simulink model "Cascaded_Rectifier_Isolated_Output"  (R2021b)
settings: Solver=VariableStepAuto  StartTime=0.0  StopTime=0.5  RelTol=1e-3
libraries: spsSeriesRLCBranchLib x41, spsUniversalBridgeLib x28, spsVoltageMeasurementLib x18, spsLinearTransformerLib x8, simulink x8, spsThreeLevelBridgeLib x7, spsACVoltageSourceLib x1, spsCurrentMeasurementLib x1, spsMeanLib x1, slpidlib x1, powerlib_extras x1, spsTHDLib x1
(part 2 of 2)

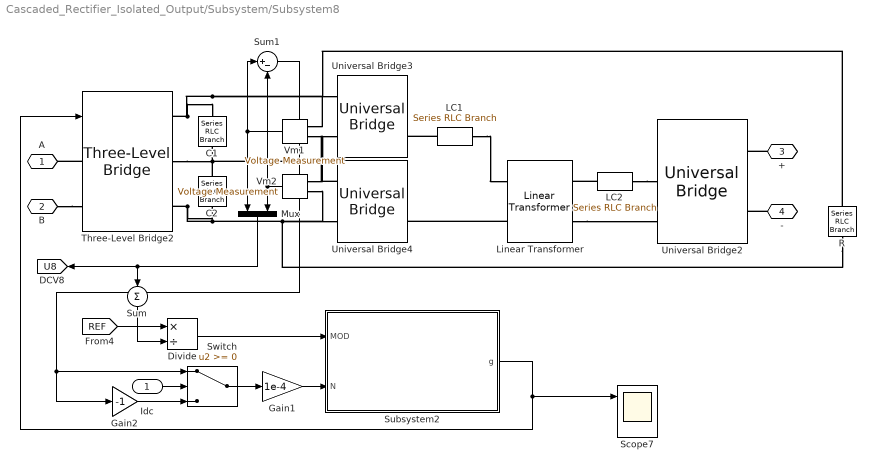
== system Cascaded_Rectifier_Isolated_Output/Subsystem/Subsystem8 ==
  Idc : Inport
  C1 : spsSeriesRLCBranchLib/Series RLC Branch  LConnTagsString=__new0  RConnTagsString=__new0  BranchType=C  Resistance=1  Inductance=7e-4  SetiL0=off  InitialCurrent=0  Capacitance=1e-3  Setx0=on  InitialVoltage=2200  Measurements=None
  C2 : spsSeriesRLCBranchLib/Series RLC Branch  LConnTagsString=__new0  RConnTagsString=__new0  BranchType=C  Resistance=1  Inductance=7e-4  SetiL0=off  InitialCurrent=0  Capacitance=1e-3  Setx0=on  InitialVoltage=2200  Measurements=None
  Divide : Product  Inputs=*/
  Gain1 : Gain  Gain=1e-4
  Gain2 : Gain  Gain=-1
  LC1 : spsSeriesRLCBranchLib/Series RLC Branch  LConnTagsString=__new0  RConnTagsString=__new0  BranchType=LC  Resistance=20  Inductance=2e-5  SetiL0=off  InitialCurrent=0  Capacitance=5.6e-7  Setx0=off  InitialVoltage=0  Measurements=None
  LC2 : spsSeriesRLCBranchLib/Series RLC Branch  LConnTagsString=__new0  RConnTagsString=__new0  BranchType=LC  Resistance=20  Inductance=2e-5  SetiL0=off  InitialCurrent=0  Capacitance=5.6e-7  Setx0=off  InitialVoltage=0  Measurements=None
  Linear Transformer : spsLinearTransformerLib/Linear Transformer  UNITS=SI  NominalPower=[ 250e3 48e3 ]  winding1=[2500 0.01 1e-6]  winding2=[2500 0.01 1e-6]  ThreeWindings=off  winding3=[3.15e+05 0.7938 0.084225]  RmLm=[1e6 1e-4]  Measurements=None  DataType=on
  Mux : Mux  Inputs=2
  R : spsSeriesRLCBranchLib/Series RLC Branch  LConnTagsString=__new0  RConnTagsString=__new0  BranchType=R  Resistance=80  Inductance=7e-4  SetiL0=off  InitialCurrent=0  Capacitance=1e-3  Setx0=off  InitialVoltage=0  Measurements=None
  Scope7 : Scope  NumInputPorts=3
  Subsystem2 : Subsystem
  Sum : Sum  Inputs=+
  Sum1 : Sum  Inputs=|+-
  Switch : Switch
  Three-Level Bridge2 : spsThreeLevelBridgeLib/Three-Level Bridge  Arms=2  SnubberResistance=1e5  SbubberCapacitance=inf  Device=IGBT / Diodes  Ron=1e-3  ForwardVoltages="[  2  2  ]"  Measurements=None
      settings: SourceProductBaseCode=PS
  Universal Bridge2 : spsUniversalBridgeLib/Universal Bridge  Arms=2  SnubberResistance=1e5  SnubberCapacitance=inf  Device=MOSFET / Diodes  Ron=1e-2  Lon=0  ForwardVoltages="[  1  1  ]"  ForwardVoltage=0  GTOparameters=[ 10e-6 , 20e-6 ]  IGBTparameters=[ 1e-6 , 2e-6 ]  Measurements=None  Measurements_2=None  converterType=Rectifier
  Universal Bridge3 : spsUniversalBridgeLib/Universal Bridge  Arms=1  SnubberResistance=1e5  SnubberCapacitance=inf  Device=MOSFET / Diodes  Ron=1e-2  Lon=0  ForwardVoltages="[  1  1  ]"  ForwardVoltage=0  GTOparameters=[ 10e-6 , 20e-6 ]  IGBTparameters=[ 1e-6 , 2e-6 ]  Measurements=None  Measurements_2=None  converterType=Rectifier
  Universal Bridge4 : spsUniversalBridgeLib/Universal Bridge  Arms=1  SnubberResistance=1e5  SnubberCapacitance=inf  Device=MOSFET / Diodes  Ron=1e-2  Lon=0  ForwardVoltages="[  1  1  ]"  ForwardVoltage=0  GTOparameters=[ 10e-6 , 20e-6 ]  IGBTparameters=[ 1e-6 , 2e-6 ]  Measurements=None  Measurements_2=None  converterType=Rectifier
  Vm1 : spsVoltageMeasurementLib/Voltage Measurement  PhasorSimulation=off  OutputType=Complex  PSBequivalent=0
  Vm2 : spsVoltageMeasurementLib/Voltage Measurement  PhasorSimulation=off  OutputType=Complex  PSBequivalent=0
  A : PMIOPort  Side=Left
  B : PMIOPort  Port=2  Side=Left
  + : PMIOPort  Port=3  Side=Right
  - : PMIOPort  Port=4  Side=Right
  tag scope: U8=global
  wires:
  Gain1/1 -> Subsystem2/2(N)
  Sum1/1 -> Switch/1, Gain2/1
  Idc/1 -> Switch/2
  Sum/1 -> Divide/2
  Vm2/1 -> Mux/2, Sum1/2
  Vm1/1 -> Sum1/1, Mux/1
  Mux/1 -> [U8], Sum/1
  Divide/1 -> Subsystem2/1(MOD)
  Subsystem2/1(g) -> Three-Level Bridge2/1, Scope7/1
  Switch/1 -> Gain1/1
  Gain2/1 -> Switch/3
  [REF] -> Divide/1
  connections:
  B/RConn1 -- Three-Level Bridge2/LConn2
  Three-Level Bridge2/LConn1 -- A/RConn1
  LC2/LConn1 -- Linear Transformer/RConn1
  LC2/RConn1 -- Universal Bridge2/LConn1
  Linear Transformer/RConn2 -- Universal Bridge2/LConn2
  LC1/RConn1 -- Linear Transformer/LConn1
  Linear Transformer/LConn2 -- Universal Bridge4/LConn1
  LC1/LConn1 -- Universal Bridge3/LConn1
  +/RConn1 -- Universal Bridge2/RConn1
  -/RConn1 -- Universal Bridge2/RConn2
  Three-Level Bridge2/RConn3 -- C2/RConn1 -- Universal Bridge4/RConn2 -- Vm2/LConn2 -- R/RConn1
  Three-Level Bridge2/RConn2 -- C1/RConn1 -- C2/LConn1 -- Universal Bridge4/RConn1 -- Vm2/LConn1 -- Universal Bridge3/RConn2 -- Vm1/LConn2
  Three-Level Bridge2/RConn1 -- Universal Bridge3/RConn1 -- Vm1/LConn1 -- R/LConn1 -- C1/LConn1

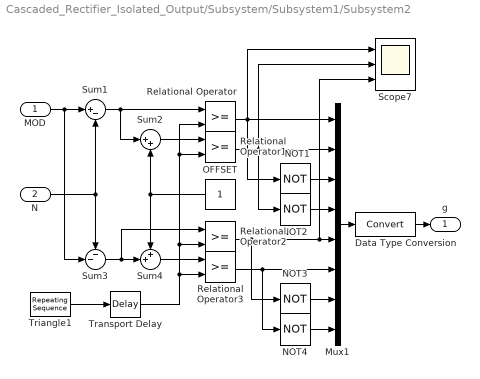
== system Cascaded_Rectifier_Isolated_Output/Subsystem/Subsystem1/Subsystem2 ==
  MOD : Inport
  N : Inport  Port=2
  Data Type Conversion : DataTypeConversion
  Mux1 : Mux  Inputs=8
  NOT{1..4} (4 alike) : Logic  Operator=NOT  IconShape=distinctive  AllPortsSameDT=off  OutDataTypeStr=boolean
  OFFSET : Constant
  Relational Operator{,1..3} (4 alike) : RelationalOperator  OutDataTypeStr=boolean  RndMeth=Nearest
  Scope7 : Scope  NumInputPorts=3
  Sum1 : Sum  Inputs=|+-
  Sum2 : Sum  Inputs=|++
  Sum3 : Sum  Inputs=--|
  Sum4 : Sum  Inputs=++|
  Transport Delay : TransportDelay  DelayTime=1/2400/8
  Triangle1 : simulink/Sources/Repeating Sequence  rep_seq_t=[0 1/1200/2 1/1200]  rep_seq_y=[0 1 0]
  g : Outport
  wires:
  Data Type Conversion/1 -> g/1
  Mux1/1 -> Data Type Conversion/1
  Sum3/1 -> Sum4/2, Relational Operator2/1
  NOT3/1 -> Mux1/7
  NOT4/1 -> Mux1/8
  Sum4/1 -> Relational Operator3/1
  OFFSET/1 -> Sum2/2, Sum4/1
  Sum2/1 -> Relational Operator1/1
  Relational Operator1/1 -> Scope7/2, Mux1/2, NOT2/1
  NOT2/1 -> Mux1/4
  NOT1/1 -> Mux1/3
  Relational Operator/1 -> Scope7/1, Mux1/1, NOT1/1
  Transport Delay/1 -> Relational Operator3/2, Relational Operator2/2, Relational Operator1/2, Relational Operator/2
  Relational Operator3/1 -> NOT4/1, Mux1/6
  Relational Operator2/1 -> NOT3/1, Scope7/3, Mux1/5
  Sum1/1 -> Relational Operator/1, Sum2/1
  MOD/1 -> Sum1/1, Sum3/2
  N/1 -> Sum1/2, Sum3/1
  Triangle1/1 -> Transport Delay/1

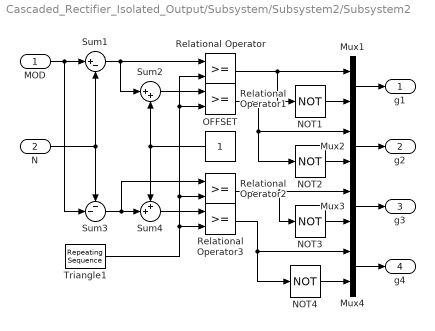
== system Cascaded_Rectifier_Isolated_Output/Subsystem/Subsystem2/Subsystem2 ==
  MOD : Inport
  N : Inport  Port=2
  Mux{1..4} (4 alike) : Mux  Inputs=2
  NOT{1..4} (4 alike) : Logic  Operator=NOT  IconShape=distinctive  AllPortsSameDT=off  OutDataTypeStr=boolean
  OFFSET : Constant
  Relational Operator{,1..3} (4 alike) : RelationalOperator  OutDataTypeStr=boolean  RndMeth=Nearest
  Sum1 : Sum  Inputs=|+-
  Sum2 : Sum  Inputs=|++
  Sum3 : Sum  Inputs=--|
  Sum4 : Sum  Inputs=++|
  Triangle1 : simulink/Sources/Repeating Sequence  rep_seq_t=[0 1/1200/2 1/1200]  rep_seq_y=[0 1 0]
  g1 : Outport
  g2 : Outport  Port=2
  g3 : Outport  Port=3
  g4 : Outport  Port=4
  wires:
  N/1 -> Sum3/1, Sum1/2
  MOD/1 -> Sum3/2, Sum1/1
  Sum1/1 -> Sum2/1, Relational Operator/1
  Relational Operator2/1 -> Mux3/1, NOT3/1
  Relational Operator3/1 -> Mux4/1, NOT4/1
  Triangle1/1 -> Relational Operator/2, Relational Operator1/2, Relational Operator2/2, Relational Operator3/2
  Relational Operator/1 -> NOT1/1, Mux1/1
  NOT2/1 -> Mux2/2
  Relational Operator1/1 -> Mux2/1, NOT2/1
  Sum2/1 -> Relational Operator1/1
  OFFSET/1 -> Sum4/1, Sum2/2
  Sum4/1 -> Relational Operator3/1
  NOT4/1 -> Mux4/2
  Sum3/1 -> Relational Operator2/1, Sum4/2
  Mux1/1 -> g1/1
  Mux2/1 -> g2/1
  Mux3/1 -> g3/1
  Mux4/1 -> g4/1
  NOT1/1 -> Mux1/2
  NOT3/1 -> Mux3/2

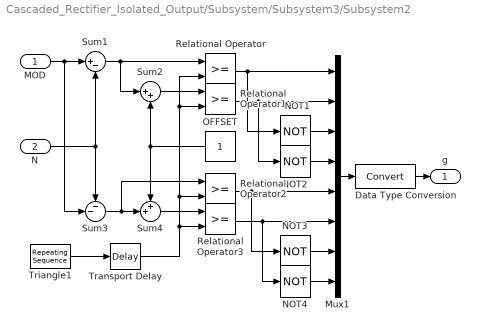
== system Cascaded_Rectifier_Isolated_Output/Subsystem/Subsystem3/Subsystem2 ==
  MOD : Inport
  N : Inport  Port=2
  Data Type Conversion : DataTypeConversion
  Mux1 : Mux  Inputs=8
  NOT{1..4} (4 alike) : Logic  Operator=NOT  IconShape=distinctive  AllPortsSameDT=off  OutDataTypeStr=boolean
  OFFSET : Constant
  Relational Operator{,1..3} (4 alike) : RelationalOperator  OutDataTypeStr=boolean  RndMeth=Nearest
  Sum1 : Sum  Inputs=|+-
  Sum2 : Sum  Inputs=|++
  Sum3 : Sum  Inputs=--|
  Sum4 : Sum  Inputs=++|
  Transport Delay : TransportDelay  DelayTime=2/2400/8
  Triangle1 : simulink/Sources/Repeating Sequence  rep_seq_t=[0 1/1200/2 1/1200]  rep_seq_y=[0 1 0]
  g : Outport
  wires:
  Triangle1/1 -> Transport Delay/1
  N/1 -> Sum3/1, Sum1/2
  MOD/1 -> Sum3/2, Sum1/1
  Sum1/1 -> Sum2/1, Relational Operator/1
  Relational Operator2/1 -> Mux1/5, NOT3/1
  Relational Operator3/1 -> Mux1/6, NOT4/1
  Transport Delay/1 -> Relational Operator/2, Relational Operator1/2, Relational Operator2/2, Relational Operator3/2
  Relational Operator/1 -> NOT1/1, Mux1/1
  NOT1/1 -> Mux1/3
  NOT2/1 -> Mux1/4
  Relational Operator1/1 -> NOT2/1, Mux1/2
  Sum2/1 -> Relational Operator1/1
  OFFSET/1 -> Sum4/1, Sum2/2
  Sum4/1 -> Relational Operator3/1
  NOT4/1 -> Mux1/8
  NOT3/1 -> Mux1/7
  Sum3/1 -> Relational Operator2/1, Sum4/2
  Mux1/1 -> Data Type Conversion/1
  Data Type Conversion/1 -> g/1

== system Cascaded_Rectifier_Isolated_Output/Subsystem/Subsystem4/Subsystem2 ==
  MOD : Inport
  N : Inport  Port=2
  Data Type Conversion : DataTypeConversion
  Mux1 : Mux  Inputs=8
  NOT{1..4} (4 alike) : Logic  Operator=NOT  IconShape=distinctive  AllPortsSameDT=off  OutDataTypeStr=boolean
  OFFSET : Constant
  Relational Operator{,1..3} (4 alike) : RelationalOperator  OutDataTypeStr=boolean  RndMeth=Nearest
  Sum1 : Sum  Inputs=|+-
  Sum2 : Sum  Inputs=|++
  Sum3 : Sum  Inputs=--|
  Sum4 : Sum  Inputs=++|
  Transport Delay : TransportDelay  DelayTime=3/2400/8
  Triangle1 : simulink/Sources/Repeating Sequence  rep_seq_t=[0 1/1200/2 1/1200]  rep_seq_y=[0 1 0]
  g : Outport
  wires:
  Data Type Conversion/1 -> g/1
  Mux1/1 -> Data Type Conversion/1
  Sum3/1 -> Sum4/2, Relational Operator2/1
  NOT3/1 -> Mux1/7
  NOT4/1 -> Mux1/8
  Sum4/1 -> Relational Operator3/1
  OFFSET/1 -> Sum2/2, Sum4/1
  Sum2/1 -> Relational Operator1/1
  Relational Operator1/1 -> Mux1/2, NOT2/1
  NOT2/1 -> Mux1/4
  NOT1/1 -> Mux1/3
  Relational Operator/1 -> Mux1/1, NOT1/1
  Transport Delay/1 -> Relational Operator3/2, Relational Operator2/2, Relational Operator1/2, Relational Operator/2
  Relational Operator3/1 -> NOT4/1, Mux1/6
  Relational Operator2/1 -> NOT3/1, Mux1/5
  Sum1/1 -> Relational Operator/1, Sum2/1
  MOD/1 -> Sum1/1, Sum3/2
  N/1 -> Sum1/2, Sum3/1
  Triangle1/1 -> Transport Delay/1

== system Cascaded_Rectifier_Isolated_Output/Subsystem/Subsystem5/Subsystem2 ==
  MOD : Inport
  N : Inport  Port=2
  Data Type Conversion : DataTypeConversion
  Mux1 : Mux  Inputs=8
  NOT{1..4} (4 alike) : Logic  Operator=NOT  IconShape=distinctive  AllPortsSameDT=off  OutDataTypeStr=boolean
  OFFSET : Constant
  Relational Operator{,1..3} (4 alike) : RelationalOperator  OutDataTypeStr=boolean  RndMeth=Nearest
  Sum1 : Sum  Inputs=|+-
  Sum2 : Sum  Inputs=|++
  Sum3 : Sum  Inputs=--|
  Sum4 : Sum  Inputs=++|
  Transport Delay : TransportDelay  DelayTime=4/2400/8
  Triangle1 : simulink/Sources/Repeating Sequence  rep_seq_t=[0 1/1200/2 1/1200]  rep_seq_y=[0 1 0]
  g : Outport
  wires:
  Triangle1/1 -> Transport Delay/1
  N/1 -> Sum3/1, Sum1/2
  MOD/1 -> Sum3/2, Sum1/1
  Sum1/1 -> Sum2/1, Relational Operator/1
  Relational Operator2/1 -> Mux1/5, NOT3/1
  Relational Operator3/1 -> Mux1/6, NOT4/1
  Transport Delay/1 -> Relational Operator/2, Relational Operator1/2, Relational Operator2/2, Relational Operator3/2
  Relational Operator/1 -> NOT1/1, Mux1/1
  NOT1/1 -> Mux1/3
  NOT2/1 -> Mux1/4
  Relational Operator1/1 -> NOT2/1, Mux1/2
  Sum2/1 -> Relational Operator1/1
  OFFSET/1 -> Sum4/1, Sum2/2
  Sum4/1 -> Relational Operator3/1
  NOT4/1 -> Mux1/8
  NOT3/1 -> Mux1/7
  Sum3/1 -> Relational Operator2/1, Sum4/2
  Mux1/1 -> Data Type Conversion/1
  Data Type Conversion/1 -> g/1

== system Cascaded_Rectifier_Isolated_Output/Subsystem/Subsystem6/Subsystem2 ==
  MOD : Inport
  N : Inport  Port=2
  Data Type Conversion : DataTypeConversion
  Mux1 : Mux  Inputs=8
  NOT{1..4} (4 alike) : Logic  Operator=NOT  IconShape=distinctive  AllPortsSameDT=off  OutDataTypeStr=boolean
  OFFSET : Constant
  Relational Operator{,1..3} (4 alike) : RelationalOperator  OutDataTypeStr=boolean  RndMeth=Nearest
  Sum1 : Sum  Inputs=|+-
  Sum2 : Sum  Inputs=|++
  Sum3 : Sum  Inputs=--|
  Sum4 : Sum  Inputs=++|
  Transport Delay : TransportDelay  DelayTime=5/2400/8
  Triangle1 : simulink/Sources/Repeating Sequence  rep_seq_t=[0 1/1200/2 1/1200]  rep_seq_y=[0 1 0]
  g : Outport
  wires:
  Data Type Conversion/1 -> g/1
  Mux1/1 -> Data Type Conversion/1
  Sum3/1 -> Sum4/2, Relational Operator2/1
  NOT3/1 -> Mux1/7
  NOT4/1 -> Mux1/8
  Sum4/1 -> Relational Operator3/1
  OFFSET/1 -> Sum2/2, Sum4/1
  Sum2/1 -> Relational Operator1/1
  Relational Operator1/1 -> Mux1/2, NOT2/1
  NOT2/1 -> Mux1/4
  NOT1/1 -> Mux1/3
  Relational Operator/1 -> Mux1/1, NOT1/1
  Transport Delay/1 -> Relational Operator3/2, Relational Operator2/2, Relational Operator1/2, Relational Operator/2
  Relational Operator3/1 -> NOT4/1, Mux1/6
  Relational Operator2/1 -> NOT3/1, Mux1/5
  Sum1/1 -> Relational Operator/1, Sum2/1
  MOD/1 -> Sum1/1, Sum3/2
  N/1 -> Sum1/2, Sum3/1
  Triangle1/1 -> Transport Delay/1

== system Cascaded_Rectifier_Isolated_Output/Subsystem/Subsystem7/Subsystem2 ==
  MOD : Inport
  N : Inport  Port=2
  Data Type Conversion : DataTypeConversion
  Mux1 : Mux  Inputs=8
  NOT{1..4} (4 alike) : Logic  Operator=NOT  IconShape=distinctive  AllPortsSameDT=off  OutDataTypeStr=boolean
  OFFSET : Constant
  Relational Operator{,1..3} (4 alike) : RelationalOperator  OutDataTypeStr=boolean  RndMeth=Nearest
  Sum1 : Sum  Inputs=|+-
  Sum2 : Sum  Inputs=|++
  Sum3 : Sum  Inputs=--|
  Sum4 : Sum  Inputs=++|
  Transport Delay : TransportDelay  DelayTime=6/2400/8
  Triangle1 : simulink/Sources/Repeating Sequence  rep_seq_t=[0 1/1200/2 1/1200]  rep_seq_y=[0 1 0]
  g : Outport
  wires:
  Triangle1/1 -> Transport Delay/1
  N/1 -> Sum3/1, Sum1/2
  MOD/1 -> Sum3/2, Sum1/1
  Sum1/1 -> Sum2/1, Relational Operator/1
  Relational Operator2/1 -> Mux1/5, NOT3/1
  Relational Operator3/1 -> Mux1/6, NOT4/1
  Transport Delay/1 -> Relational Operator/2, Relational Operator1/2, Relational Operator2/2, Relational Operator3/2
  Relational Operator/1 -> NOT1/1, Mux1/1
  NOT1/1 -> Mux1/3
  NOT2/1 -> Mux1/4
  Relational Operator1/1 -> NOT2/1, Mux1/2
  Sum2/1 -> Relational Operator1/1
  OFFSET/1 -> Sum4/1, Sum2/2
  Sum4/1 -> Relational Operator3/1
  NOT4/1 -> Mux1/8
  NOT3/1 -> Mux1/7
  Sum3/1 -> Relational Operator2/1, Sum4/2
  Mux1/1 -> Data Type Conversion/1
  Data Type Conversion/1 -> g/1

== system Cascaded_Rectifier_Isolated_Output/Subsystem/Subsystem8/Subsystem2 ==
  MOD : Inport
  N : Inport  Port=2
  Data Type Conversion : DataTypeConversion
  Mux1 : Mux  Inputs=8
  NOT{1..4} (4 alike) : Logic  Operator=NOT  IconShape=distinctive  AllPortsSameDT=off  OutDataTypeStr=boolean
  OFFSET : Constant
  Relational Operator{,1..3} (4 alike) : RelationalOperator  OutDataTypeStr=boolean  RndMeth=Nearest
  Sum1 : Sum  Inputs=|+-
  Sum2 : Sum  Inputs=|++
  Sum3 : Sum  Inputs=--|
  Sum4 : Sum  Inputs=++|
  Transport Delay : TransportDelay  DelayTime=7/2400/8
  Triangle1 : simulink/Sources/Repeating Sequence  rep_seq_t=[0 1/1200/2 1/1200]  rep_seq_y=[0 1 0]
  g : Outport
  wires:
  Data Type Conversion/1 -> g/1
  Mux1/1 -> Data Type Conversion/1
  Sum3/1 -> Sum4/2, Relational Operator2/1
  NOT3/1 -> Mux1/7
  NOT4/1 -> Mux1/8
  Sum4/1 -> Relational Operator3/1
  OFFSET/1 -> Sum2/2, Sum4/1
  Sum2/1 -> Relational Operator1/1
  Relational Operator1/1 -> Mux1/2, NOT2/1
  NOT2/1 -> Mux1/4
  NOT1/1 -> Mux1/3
  Relational Operator/1 -> Mux1/1, NOT1/1
  Transport Delay/1 -> Relational Operator3/2, Relational Operator2/2, Relational Operator1/2, Relational Operator/2
  Relational Operator3/1 -> NOT4/1, Mux1/6
  Relational Operator2/1 -> NOT3/1, Mux1/5
  Sum1/1 -> Relational Operator/1, Sum2/1
  MOD/1 -> Sum1/1, Sum3/2
  N/1 -> Sum1/2, Sum3/1
  Triangle1/1 -> Transport Delay/1

== matlab function Cascaded_Rectifier_Isolated_Output/PF ==
  data: P input; PF output; Q input; iTHD input
function PF = fcn(P,Q,iTHD)
% This block supports an embeddable subset of the MATLAB language.
% See the help menu for details. 
PF=(P/sqrt(P*P+Q*Q))/(sqrt(1+iTHD*iTHD));
